simulink model "A1_1"  (R2018b)
settings: Solver=ode45  StartTime=0.0  StopTime=40  RelTol=1e-3
settings Model: Creator=lenovo  LastModifiedBy=lenovo

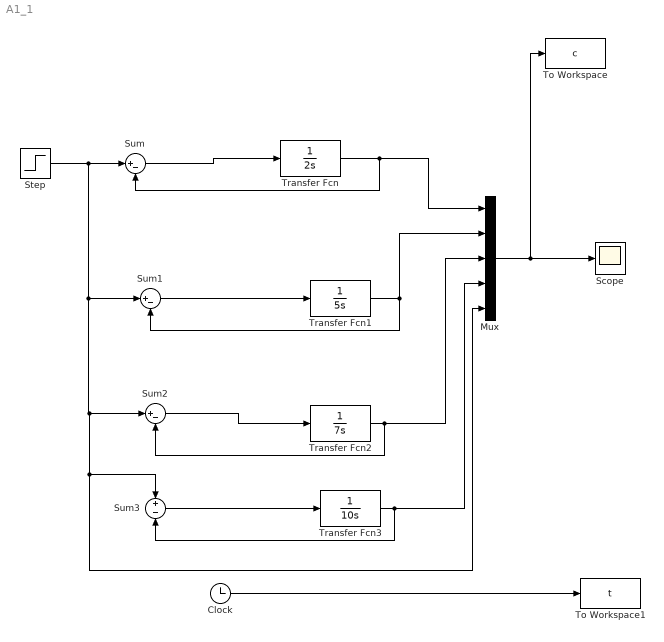
== system A1_1 ==
  Clock : Clock
  Mux : Mux  Inputs=5
  Scope : Scope
  Step : Step  SampleTime=0
  Sum : Sum  Inputs=|+-
  Sum1 : Sum  Inputs=|+-
  Sum2 : Sum  Inputs=|+-
  Sum3 : Sum  Inputs=+-
  To Workspace : ToWorkspace  VariableName=c  SampleTime=-1
  To Workspace1 : ToWorkspace  VariableName=t  SampleTime=-1
  Transfer Fcn : TransferFcn  Denominator=[2 0]
  Transfer Fcn1 : TransferFcn  Denominator=[5 0]
  Transfer Fcn2 : TransferFcn  Denominator=[7 0]
  Transfer Fcn3 : TransferFcn  Denominator=[10 0]
  wires:
  Step/1 -> Sum2/1, Sum3/1, Mux/5, Sum1/1, Sum/1
  Sum/1 -> Transfer Fcn/1
  Sum1/1 -> Transfer Fcn1/1
  Sum2/1 -> Transfer Fcn2/1
  Clock/1 -> To Workspace1/1
  Transfer Fcn/1 -> Mux/1, Sum/2
  Transfer Fcn1/1 -> Sum1/2, Mux/2
  Transfer Fcn2/1 -> Mux/3, Sum2/2
  Mux/1 -> To Workspace/1, Scope/1
  Sum3/1 -> Transfer Fcn3/1
  Transfer Fcn3/1 -> Mux/4, Sum3/2
